simulink model "rolling_contact_36_example"  (R2026b)
settings: Solver=VariableStepAuto  StopTime=5
undefined symbols (not defined in the file): f_rr, k_gx, k_gy, k_x, m_wheel, miu_p, miu_s, mu_slide, mu_stick, omega_rr_eps, r_wheel, sgn, v_gx_max, v_gy_max, vLimit, X, Y, Z
libraries: nesl_utility x225, sm_lib x156, simulink x146, simulink_extras x36
(part 3 of 11)

== system rolling_contact_36_example/36-Point Sliding Contact Model/Body Contact 1 ==
  note: Planar Ground Interaction Model
  " Body Actuator" : nesl_utility/Simulink-PS Converter  PhysicalDomain=network_engine_domain  SubClassName=ps_input  LeftPortType=input  RightPortType=output  PseudoPeriodic=off  Frequencies=[]  NoiseDistribution=none  NoiseParameters=[]  Unit=N  AffineConversion=off  FilteringAndDerivatives=zero  SimscapeFilterOrder=1  InputFilterTimeConstant=.001  UdotUserProvided=0
  " Body Actuator1" : nesl_utility/Simulink-PS Converter  PhysicalDomain=network_engine_domain  SubClassName=ps_input  LeftPortType=input  RightPortType=output  PseudoPeriodic=off  Frequencies=[]  NoiseDistribution=none  NoiseParameters=[]  Unit=N  AffineConversion=off  FilteringAndDerivatives=zero  SimscapeFilterOrder=1  InputFilterTimeConstant=.001  UdotUserProvided=0
  External Force and Torque : sm_lib/Forces and Torques/External Force and Torque  EnableForceX=on  EnableForceY=on  EnableForceZ=off  EnableForce=off  ForceResolutionFrame=World  EnableTorqueX=off  EnableTorqueY=off  EnableTorqueZ=off  EnableTorque=off  TorqueResolutionFrame=AttachedFrame
  Frame Sensor : sm_lib/Frames and Transforms/Transform Sensor  ObservationFrame=World  ExpressedInFrame=World  RotationSequence=XYX  SenseAngle=off  SenseAxis=off  SenseQ=off  SenseR=off  SenseRotationSequence=off  SenseOmegaX=off  SenseOmegaY=off  SenseOmegaZ=off  SenseOmega=off  SenseQDot=off  SenseRDot=off  SenseRotationSequenceDot=off  SenseAlphaX=off  SenseAlphaY=off  SenseAlphaZ=off  SenseAlpha=off  SenseQDDot=off  SenseRDDot=off  SenseX=on  SenseY=on  SenseZ=off  SenseXYZ=off  SenseRad=off  SenseAzim=off  SenseDist=off  SenseInc=off  SenseXDot=on  SenseYDot=on  SenseZDot=off  SenseXYZDot=off  SenseRadDot=off  SenseAzimDot=off  SenseDistDot=off  SenseIncDot=off  SenseXDDot=off  SenseYDDot=off  SenseZDDot=off  SenseXYZDDot=off  SenseRadDDot=off  SenseAzimDDot=off  SenseDistDDot=off  SenseIncDDot=off
  Ground Friction Model : Subsystem
  PS-Simulink Converter : nesl_utility/PS-Simulink Converter  PhysicalDomain=network_engine_domain  SubClassName=ps_output  LeftPortType=input  RightPortType=output  PseudoPeriodic=off  Frequencies=[]  VectorFormat=1-D array  Unit=m  AffineConversion=off
  PS-Simulink Converter1 : nesl_utility/PS-Simulink Converter  PhysicalDomain=network_engine_domain  SubClassName=ps_output  LeftPortType=input  RightPortType=output  PseudoPeriodic=off  Frequencies=[]  VectorFormat=1-D array  Unit=m  AffineConversion=off
  PS-Simulink Converter2 : nesl_utility/PS-Simulink Converter  PhysicalDomain=network_engine_domain  SubClassName=ps_output  LeftPortType=input  RightPortType=output  PseudoPeriodic=off  Frequencies=[]  VectorFormat=1-D array  Unit=m/s  AffineConversion=off
  PS-Simulink Converter3 : nesl_utility/PS-Simulink Converter  PhysicalDomain=network_engine_domain  SubClassName=ps_output  LeftPortType=input  RightPortType=output  PseudoPeriodic=off  Frequencies=[]  VectorFormat=1-D array  Unit=m/s  AffineConversion=off
  Sum : Sum  Inputs=-+|
  Terminator : Terminator
  World Frame : sm_lib/Frames and Transforms/World Frame
  contact sensor : simulink/Logic and Bit Operations/Compare To Zero  relop=<=  OutDataTypeStr=boolean
  yGround : Constant  Value=0
  F : PMIOPort  Side=Left
  Fx patch [N] : Outport
  Fy patch [N] : Outport  Port=2
  wires:
  PS-Simulink Converter2/1 -> Ground Friction Model/4(vx [m/s])
  PS-Simulink Converter/1 -> Ground Friction Model/3(x [m])
  PS-Simulink Converter3/1 -> Ground Friction Model/2(vy [m/s])
  PS-Simulink Converter1/1 -> Sum/2
  Sum/1 -> contact sensor/1, Ground Friction Model/1(dy [m])
  yGround/1 -> Sum/1
  contact sensor/1 -> Ground Friction Model/Enable
  Ground Friction Model/1(Fy_Ground[N]) -> " Body Actuator1"/1, Fy patch [N]/1
  Ground Friction Model/2(Fx_Friction [N]) -> " Body Actuator"/1, Fx patch [N]/1
  Ground Friction Model/3(Stiction!) -> Terminator/1
  connections:
  World Frame/RConn1 -- Frame Sensor/LConn1
  PS-Simulink Converter2/LConn1 -- Frame Sensor/RConn4
  PS-Simulink Converter1/LConn1 -- Frame Sensor/RConn3
  Frame Sensor/RConn2 -- PS-Simulink Converter/LConn1
  PS-Simulink Converter3/LConn1 -- Frame Sensor/RConn5
  External Force and Torque/RConn1 -- Frame Sensor/RConn1 -- F/RConn1
  External Force and Torque/LConn2 -- " Body Actuator1"/RConn1
  External Force and Torque/LConn1 -- " Body Actuator"/RConn1

== system rolling_contact_36_example/36-Point Sliding Contact Model/Body Contact 10 ==
  note: Planar Ground Interaction Model
  " Body Actuator" : nesl_utility/Simulink-PS Converter  PhysicalDomain=network_engine_domain  SubClassName=ps_input  LeftPortType=input  RightPortType=output  PseudoPeriodic=off  Frequencies=[]  NoiseDistribution=none  NoiseParameters=[]  Unit=N  AffineConversion=off  FilteringAndDerivatives=zero  SimscapeFilterOrder=1  InputFilterTimeConstant=.001  UdotUserProvided=0
  " Body Actuator1" : nesl_utility/Simulink-PS Converter  PhysicalDomain=network_engine_domain  SubClassName=ps_input  LeftPortType=input  RightPortType=output  PseudoPeriodic=off  Frequencies=[]  NoiseDistribution=none  NoiseParameters=[]  Unit=N  AffineConversion=off  FilteringAndDerivatives=zero  SimscapeFilterOrder=1  InputFilterTimeConstant=.001  UdotUserProvided=0
  External Force and Torque : sm_lib/Forces and Torques/External Force and Torque  EnableForceX=on  EnableForceY=on  EnableForceZ=off  EnableForce=off  ForceResolutionFrame=World  EnableTorqueX=off  EnableTorqueY=off  EnableTorqueZ=off  EnableTorque=off  TorqueResolutionFrame=AttachedFrame
  Frame Sensor : sm_lib/Frames and Transforms/Transform Sensor  ObservationFrame=World  ExpressedInFrame=World  RotationSequence=XYX  SenseAngle=off  SenseAxis=off  SenseQ=off  SenseR=off  SenseRotationSequence=off  SenseOmegaX=off  SenseOmegaY=off  SenseOmegaZ=off  SenseOmega=off  SenseQDot=off  SenseRDot=off  SenseRotationSequenceDot=off  SenseAlphaX=off  SenseAlphaY=off  SenseAlphaZ=off  SenseAlpha=off  SenseQDDot=off  SenseRDDot=off  SenseX=on  SenseY=on  SenseZ=off  SenseXYZ=off  SenseRad=off  SenseAzim=off  SenseDist=off  SenseInc=off  SenseXDot=on  SenseYDot=on  SenseZDot=off  SenseXYZDot=off  SenseRadDot=off  SenseAzimDot=off  SenseDistDot=off  SenseIncDot=off  SenseXDDot=off  SenseYDDot=off  SenseZDDot=off  SenseXYZDDot=off  SenseRadDDot=off  SenseAzimDDot=off  SenseDistDDot=off  SenseIncDDot=off
  Ground Friction Model : Subsystem
  PS-Simulink Converter : nesl_utility/PS-Simulink Converter  PhysicalDomain=network_engine_domain  SubClassName=ps_output  LeftPortType=input  RightPortType=output  PseudoPeriodic=off  Frequencies=[]  VectorFormat=1-D array  Unit=m  AffineConversion=off
  PS-Simulink Converter1 : nesl_utility/PS-Simulink Converter  PhysicalDomain=network_engine_domain  SubClassName=ps_output  LeftPortType=input  RightPortType=output  PseudoPeriodic=off  Frequencies=[]  VectorFormat=1-D array  Unit=m  AffineConversion=off
  PS-Simulink Converter2 : nesl_utility/PS-Simulink Converter  PhysicalDomain=network_engine_domain  SubClassName=ps_output  LeftPortType=input  RightPortType=output  PseudoPeriodic=off  Frequencies=[]  VectorFormat=1-D array  Unit=m/s  AffineConversion=off
  PS-Simulink Converter3 : nesl_utility/PS-Simulink Converter  PhysicalDomain=network_engine_domain  SubClassName=ps_output  LeftPortType=input  RightPortType=output  PseudoPeriodic=off  Frequencies=[]  VectorFormat=1-D array  Unit=m/s  AffineConversion=off
  Sum : Sum  Inputs=-+|
  Terminator : Terminator
  World Frame : sm_lib/Frames and Transforms/World Frame
  contact sensor : simulink/Logic and Bit Operations/Compare To Zero  relop=<=  OutDataTypeStr=boolean
  yGround : Constant  Value=0
  F : PMIOPort  Side=Left
  Fx patch [N] : Outport
  Fy patch [N] : Outport  Port=2
  wires:
  Ground Friction Model/3(Stiction!) -> Terminator/1
  Ground Friction Model/2(Fx_Friction [N]) -> " Body Actuator"/1, Fx patch [N]/1
  Ground Friction Model/1(Fy_Ground[N]) -> " Body Actuator1"/1, Fy patch [N]/1
  contact sensor/1 -> Ground Friction Model/Enable
  yGround/1 -> Sum/1
  Sum/1 -> Ground Friction Model/1(dy [m]), contact sensor/1
  PS-Simulink Converter1/1 -> Sum/2
  PS-Simulink Converter3/1 -> Ground Friction Model/2(vy [m/s])
  PS-Simulink Converter/1 -> Ground Friction Model/3(x [m])
  PS-Simulink Converter2/1 -> Ground Friction Model/4(vx [m/s])
  connections:
  External Force and Torque/LConn1 -- " Body Actuator"/RConn1
  External Force and Torque/LConn2 -- " Body Actuator1"/RConn1
  F/RConn1 -- Frame Sensor/RConn1 -- External Force and Torque/RConn1
  PS-Simulink Converter3/LConn1 -- Frame Sensor/RConn5
  Frame Sensor/RConn2 -- PS-Simulink Converter/LConn1
  PS-Simulink Converter1/LConn1 -- Frame Sensor/RConn3
  PS-Simulink Converter2/LConn1 -- Frame Sensor/RConn4
  World Frame/RConn1 -- Frame Sensor/LConn1

== system rolling_contact_36_example/36-Point Sliding Contact Model/Body Contact 11 ==
  note: Planar Ground Interaction Model
  " Body Actuator" : nesl_utility/Simulink-PS Converter  PhysicalDomain=network_engine_domain  SubClassName=ps_input  LeftPortType=input  RightPortType=output  PseudoPeriodic=off  Frequencies=[]  NoiseDistribution=none  NoiseParameters=[]  Unit=N  AffineConversion=off  FilteringAndDerivatives=zero  SimscapeFilterOrder=1  InputFilterTimeConstant=.001  UdotUserProvided=0
  " Body Actuator1" : nesl_utility/Simulink-PS Converter  PhysicalDomain=network_engine_domain  SubClassName=ps_input  LeftPortType=input  RightPortType=output  PseudoPeriodic=off  Frequencies=[]  NoiseDistribution=none  NoiseParameters=[]  Unit=N  AffineConversion=off  FilteringAndDerivatives=zero  SimscapeFilterOrder=1  InputFilterTimeConstant=.001  UdotUserProvided=0
  External Force and Torque : sm_lib/Forces and Torques/External Force and Torque  EnableForceX=on  EnableForceY=on  EnableForceZ=off  EnableForce=off  ForceResolutionFrame=World  EnableTorqueX=off  EnableTorqueY=off  EnableTorqueZ=off  EnableTorque=off  TorqueResolutionFrame=AttachedFrame
  Frame Sensor : sm_lib/Frames and Transforms/Transform Sensor  ObservationFrame=World  ExpressedInFrame=World  RotationSequence=XYX  SenseAngle=off  SenseAxis=off  SenseQ=off  SenseR=off  SenseRotationSequence=off  SenseOmegaX=off  SenseOmegaY=off  SenseOmegaZ=off  SenseOmega=off  SenseQDot=off  SenseRDot=off  SenseRotationSequenceDot=off  SenseAlphaX=off  SenseAlphaY=off  SenseAlphaZ=off  SenseAlpha=off  SenseQDDot=off  SenseRDDot=off  SenseX=on  SenseY=on  SenseZ=off  SenseXYZ=off  SenseRad=off  SenseAzim=off  SenseDist=off  SenseInc=off  SenseXDot=on  SenseYDot=on  SenseZDot=off  SenseXYZDot=off  SenseRadDot=off  SenseAzimDot=off  SenseDistDot=off  SenseIncDot=off  SenseXDDot=off  SenseYDDot=off  SenseZDDot=off  SenseXYZDDot=off  SenseRadDDot=off  SenseAzimDDot=off  SenseDistDDot=off  SenseIncDDot=off
  Ground Friction Model : Subsystem
  PS-Simulink Converter : nesl_utility/PS-Simulink Converter  PhysicalDomain=network_engine_domain  SubClassName=ps_output  LeftPortType=input  RightPortType=output  PseudoPeriodic=off  Frequencies=[]  VectorFormat=1-D array  Unit=m  AffineConversion=off
  PS-Simulink Converter1 : nesl_utility/PS-Simulink Converter  PhysicalDomain=network_engine_domain  SubClassName=ps_output  LeftPortType=input  RightPortType=output  PseudoPeriodic=off  Frequencies=[]  VectorFormat=1-D array  Unit=m  AffineConversion=off
  PS-Simulink Converter2 : nesl_utility/PS-Simulink Converter  PhysicalDomain=network_engine_domain  SubClassName=ps_output  LeftPortType=input  RightPortType=output  PseudoPeriodic=off  Frequencies=[]  VectorFormat=1-D array  Unit=m/s  AffineConversion=off
  PS-Simulink Converter3 : nesl_utility/PS-Simulink Converter  PhysicalDomain=network_engine_domain  SubClassName=ps_output  LeftPortType=input  RightPortType=output  PseudoPeriodic=off  Frequencies=[]  VectorFormat=1-D array  Unit=m/s  AffineConversion=off
  Sum : Sum  Inputs=-+|
  Terminator : Terminator
  World Frame : sm_lib/Frames and Transforms/World Frame
  contact sensor : simulink/Logic and Bit Operations/Compare To Zero  relop=<=  OutDataTypeStr=boolean
  yGround : Constant  Value=0
  F : PMIOPort  Side=Left
  Fx patch [N] : Outport
  Fy patch [N] : Outport  Port=2
  wires:
  PS-Simulink Converter2/1 -> Ground Friction Model/4(vx [m/s])
  PS-Simulink Converter/1 -> Ground Friction Model/3(x [m])
  PS-Simulink Converter3/1 -> Ground Friction Model/2(vy [m/s])
  PS-Simulink Converter1/1 -> Sum/2
  Sum/1 -> contact sensor/1, Ground Friction Model/1(dy [m])
  yGround/1 -> Sum/1
  contact sensor/1 -> Ground Friction Model/Enable
  Ground Friction Model/1(Fy_Ground[N]) -> " Body Actuator1"/1, Fy patch [N]/1
  Ground Friction Model/2(Fx_Friction [N]) -> " Body Actuator"/1, Fx patch [N]/1
  Ground Friction Model/3(Stiction!) -> Terminator/1
  connections:
  World Frame/RConn1 -- Frame Sensor/LConn1
  PS-Simulink Converter2/LConn1 -- Frame Sensor/RConn4
  PS-Simulink Converter1/LConn1 -- Frame Sensor/RConn3
  Frame Sensor/RConn2 -- PS-Simulink Converter/LConn1
  PS-Simulink Converter3/LConn1 -- Frame Sensor/RConn5
  External Force and Torque/RConn1 -- Frame Sensor/RConn1 -- F/RConn1
  External Force and Torque/LConn2 -- " Body Actuator1"/RConn1
  External Force and Torque/LConn1 -- " Body Actuator"/RConn1

== system rolling_contact_36_example/36-Point Sliding Contact Model/Body Contact 12 ==
  note: Planar Ground Interaction Model
  " Body Actuator" : nesl_utility/Simulink-PS Converter  PhysicalDomain=network_engine_domain  SubClassName=ps_input  LeftPortType=input  RightPortType=output  PseudoPeriodic=off  Frequencies=[]  NoiseDistribution=none  NoiseParameters=[]  Unit=N  AffineConversion=off  FilteringAndDerivatives=zero  SimscapeFilterOrder=1  InputFilterTimeConstant=.001  UdotUserProvided=0
  " Body Actuator1" : nesl_utility/Simulink-PS Converter  PhysicalDomain=network_engine_domain  SubClassName=ps_input  LeftPortType=input  RightPortType=output  PseudoPeriodic=off  Frequencies=[]  NoiseDistribution=none  NoiseParameters=[]  Unit=N  AffineConversion=off  FilteringAndDerivatives=zero  SimscapeFilterOrder=1  InputFilterTimeConstant=.001  UdotUserProvided=0
  External Force and Torque : sm_lib/Forces and Torques/External Force and Torque  EnableForceX=on  EnableForceY=on  EnableForceZ=off  EnableForce=off  ForceResolutionFrame=World  EnableTorqueX=off  EnableTorqueY=off  EnableTorqueZ=off  EnableTorque=off  TorqueResolutionFrame=AttachedFrame
  Frame Sensor : sm_lib/Frames and Transforms/Transform Sensor  ObservationFrame=World  ExpressedInFrame=World  RotationSequence=XYX  SenseAngle=off  SenseAxis=off  SenseQ=off  SenseR=off  SenseRotationSequence=off  SenseOmegaX=off  SenseOmegaY=off  SenseOmegaZ=off  SenseOmega=off  SenseQDot=off  SenseRDot=off  SenseRotationSequenceDot=off  SenseAlphaX=off  SenseAlphaY=off  SenseAlphaZ=off  SenseAlpha=off  SenseQDDot=off  SenseRDDot=off  SenseX=on  SenseY=on  SenseZ=off  SenseXYZ=off  SenseRad=off  SenseAzim=off  SenseDist=off  SenseInc=off  SenseXDot=on  SenseYDot=on  SenseZDot=off  SenseXYZDot=off  SenseRadDot=off  SenseAzimDot=off  SenseDistDot=off  SenseIncDot=off  SenseXDDot=off  SenseYDDot=off  SenseZDDot=off  SenseXYZDDot=off  SenseRadDDot=off  SenseAzimDDot=off  SenseDistDDot=off  SenseIncDDot=off
  Ground Friction Model : Subsystem
  PS-Simulink Converter : nesl_utility/PS-Simulink Converter  PhysicalDomain=network_engine_domain  SubClassName=ps_output  LeftPortType=input  RightPortType=output  PseudoPeriodic=off  Frequencies=[]  VectorFormat=1-D array  Unit=m  AffineConversion=off
  PS-Simulink Converter1 : nesl_utility/PS-Simulink Converter  PhysicalDomain=network_engine_domain  SubClassName=ps_output  LeftPortType=input  RightPortType=output  PseudoPeriodic=off  Frequencies=[]  VectorFormat=1-D array  Unit=m  AffineConversion=off
  PS-Simulink Converter2 : nesl_utility/PS-Simulink Converter  PhysicalDomain=network_engine_domain  SubClassName=ps_output  LeftPortType=input  RightPortType=output  PseudoPeriodic=off  Frequencies=[]  VectorFormat=1-D array  Unit=m/s  AffineConversion=off
  PS-Simulink Converter3 : nesl_utility/PS-Simulink Converter  PhysicalDomain=network_engine_domain  SubClassName=ps_output  LeftPortType=input  RightPortType=output  PseudoPeriodic=off  Frequencies=[]  VectorFormat=1-D array  Unit=m/s  AffineConversion=off
  Sum : Sum  Inputs=-+|
  Terminator : Terminator
  World Frame : sm_lib/Frames and Transforms/World Frame
  contact sensor : simulink/Logic and Bit Operations/Compare To Zero  relop=<=  OutDataTypeStr=boolean
  yGround : Constant  Value=0
  F : PMIOPort  Side=Left
  Fx patch [N] : Outport
  Fy patch [N] : Outport  Port=2
  wires:
  Ground Friction Model/3(Stiction!) -> Terminator/1
  Ground Friction Model/2(Fx_Friction [N]) -> " Body Actuator"/1, Fx patch [N]/1
  Ground Friction Model/1(Fy_Ground[N]) -> " Body Actuator1"/1, Fy patch [N]/1
  contact sensor/1 -> Ground Friction Model/Enable
  yGround/1 -> Sum/1
  Sum/1 -> Ground Friction Model/1(dy [m]), contact sensor/1
  PS-Simulink Converter1/1 -> Sum/2
  PS-Simulink Converter3/1 -> Ground Friction Model/2(vy [m/s])
  PS-Simulink Converter/1 -> Ground Friction Model/3(x [m])
  PS-Simulink Converter2/1 -> Ground Friction Model/4(vx [m/s])
  connections:
  External Force and Torque/LConn1 -- " Body Actuator"/RConn1
  External Force and Torque/LConn2 -- " Body Actuator1"/RConn1
  F/RConn1 -- Frame Sensor/RConn1 -- External Force and Torque/RConn1
  PS-Simulink Converter3/LConn1 -- Frame Sensor/RConn5
  Frame Sensor/RConn2 -- PS-Simulink Converter/LConn1
  PS-Simulink Converter1/LConn1 -- Frame Sensor/RConn3
  PS-Simulink Converter2/LConn1 -- Frame Sensor/RConn4
  World Frame/RConn1 -- Frame Sensor/LConn1

== system rolling_contact_36_example/36-Point Sliding Contact Model/Body Contact 13 ==
  note: Planar Ground Interaction Model
  " Body Actuator" : nesl_utility/Simulink-PS Converter  PhysicalDomain=network_engine_domain  SubClassName=ps_input  LeftPortType=input  RightPortType=output  PseudoPeriodic=off  Frequencies=[]  NoiseDistribution=none  NoiseParameters=[]  Unit=N  AffineConversion=off  FilteringAndDerivatives=zero  SimscapeFilterOrder=1  InputFilterTimeConstant=.001  UdotUserProvided=0
  " Body Actuator1" : nesl_utility/Simulink-PS Converter  PhysicalDomain=network_engine_domain  SubClassName=ps_input  LeftPortType=input  RightPortType=output  PseudoPeriodic=off  Frequencies=[]  NoiseDistribution=none  NoiseParameters=[]  Unit=N  AffineConversion=off  FilteringAndDerivatives=zero  SimscapeFilterOrder=1  InputFilterTimeConstant=.001  UdotUserProvided=0
  External Force and Torque : sm_lib/Forces and Torques/External Force and Torque  EnableForceX=on  EnableForceY=on  EnableForceZ=off  EnableForce=off  ForceResolutionFrame=World  EnableTorqueX=off  EnableTorqueY=off  EnableTorqueZ=off  EnableTorque=off  TorqueResolutionFrame=AttachedFrame
  Frame Sensor : sm_lib/Frames and Transforms/Transform Sensor  ObservationFrame=World  ExpressedInFrame=World  RotationSequence=XYX  SenseAngle=off  SenseAxis=off  SenseQ=off  SenseR=off  SenseRotationSequence=off  SenseOmegaX=off  SenseOmegaY=off  SenseOmegaZ=off  SenseOmega=off  SenseQDot=off  SenseRDot=off  SenseRotationSequenceDot=off  SenseAlphaX=off  SenseAlphaY=off  SenseAlphaZ=off  SenseAlpha=off  SenseQDDot=off  SenseRDDot=off  SenseX=on  SenseY=on  SenseZ=off  SenseXYZ=off  SenseRad=off  SenseAzim=off  SenseDist=off  SenseInc=off  SenseXDot=on  SenseYDot=on  SenseZDot=off  SenseXYZDot=off  SenseRadDot=off  SenseAzimDot=off  SenseDistDot=off  SenseIncDot=off  SenseXDDot=off  SenseYDDot=off  SenseZDDot=off  SenseXYZDDot=off  SenseRadDDot=off  SenseAzimDDot=off  SenseDistDDot=off  SenseIncDDot=off
  Ground Friction Model : Subsystem
  PS-Simulink Converter : nesl_utility/PS-Simulink Converter  PhysicalDomain=network_engine_domain  SubClassName=ps_output  LeftPortType=input  RightPortType=output  PseudoPeriodic=off  Frequencies=[]  VectorFormat=1-D array  Unit=m  AffineConversion=off
  PS-Simulink Converter1 : nesl_utility/PS-Simulink Converter  PhysicalDomain=network_engine_domain  SubClassName=ps_output  LeftPortType=input  RightPortType=output  PseudoPeriodic=off  Frequencies=[]  VectorFormat=1-D array  Unit=m  AffineConversion=off
  PS-Simulink Converter2 : nesl_utility/PS-Simulink Converter  PhysicalDomain=network_engine_domain  SubClassName=ps_output  LeftPortType=input  RightPortType=output  PseudoPeriodic=off  Frequencies=[]  VectorFormat=1-D array  Unit=m/s  AffineConversion=off
  PS-Simulink Converter3 : nesl_utility/PS-Simulink Converter  PhysicalDomain=network_engine_domain  SubClassName=ps_output  LeftPortType=input  RightPortType=output  PseudoPeriodic=off  Frequencies=[]  VectorFormat=1-D array  Unit=m/s  AffineConversion=off
  Sum : Sum  Inputs=-+|
  Terminator : Terminator
  World Frame : sm_lib/Frames and Transforms/World Frame
  contact sensor : simulink/Logic and Bit Operations/Compare To Zero  relop=<=  OutDataTypeStr=boolean
  yGround : Constant  Value=0
  F : PMIOPort  Side=Left
  Fx patch [N] : Outport
  Fy patch [N] : Outport  Port=2
  wires:
  PS-Simulink Converter2/1 -> Ground Friction Model/4(vx [m/s])
  PS-Simulink Converter/1 -> Ground Friction Model/3(x [m])
  PS-Simulink Converter3/1 -> Ground Friction Model/2(vy [m/s])
  PS-Simulink Converter1/1 -> Sum/2
  Sum/1 -> contact sensor/1, Ground Friction Model/1(dy [m])
  yGround/1 -> Sum/1
  contact sensor/1 -> Ground Friction Model/Enable
  Ground Friction Model/1(Fy_Ground[N]) -> " Body Actuator1"/1, Fy patch [N]/1
  Ground Friction Model/2(Fx_Friction [N]) -> " Body Actuator"/1, Fx patch [N]/1
  Ground Friction Model/3(Stiction!) -> Terminator/1
  connections:
  World Frame/RConn1 -- Frame Sensor/LConn1
  PS-Simulink Converter2/LConn1 -- Frame Sensor/RConn4
  PS-Simulink Converter1/LConn1 -- Frame Sensor/RConn3
  Frame Sensor/RConn2 -- PS-Simulink Converter/LConn1
  PS-Simulink Converter3/LConn1 -- Frame Sensor/RConn5
  External Force and Torque/RConn1 -- Frame Sensor/RConn1 -- F/RConn1
  External Force and Torque/LConn2 -- " Body Actuator1"/RConn1
  External Force and Torque/LConn1 -- " Body Actuator"/RConn1

== system rolling_contact_36_example/36-Point Sliding Contact Model/Body Contact 14 ==
  note: Planar Ground Interaction Model
  " Body Actuator" : nesl_utility/Simulink-PS Converter  PhysicalDomain=network_engine_domain  SubClassName=ps_input  LeftPortType=input  RightPortType=output  PseudoPeriodic=off  Frequencies=[]  NoiseDistribution=none  NoiseParameters=[]  Unit=N  AffineConversion=off  FilteringAndDerivatives=zero  SimscapeFilterOrder=1  InputFilterTimeConstant=.001  UdotUserProvided=0
  " Body Actuator1" : nesl_utility/Simulink-PS Converter  PhysicalDomain=network_engine_domain  SubClassName=ps_input  LeftPortType=input  RightPortType=output  PseudoPeriodic=off  Frequencies=[]  NoiseDistribution=none  NoiseParameters=[]  Unit=N  AffineConversion=off  FilteringAndDerivatives=zero  SimscapeFilterOrder=1  InputFilterTimeConstant=.001  UdotUserProvided=0
  External Force and Torque : sm_lib/Forces and Torques/External Force and Torque  EnableForceX=on  EnableForceY=on  EnableForceZ=off  EnableForce=off  ForceResolutionFrame=World  EnableTorqueX=off  EnableTorqueY=off  EnableTorqueZ=off  EnableTorque=off  TorqueResolutionFrame=AttachedFrame
  Frame Sensor : sm_lib/Frames and Transforms/Transform Sensor  ObservationFrame=World  ExpressedInFrame=World  RotationSequence=XYX  SenseAngle=off  SenseAxis=off  SenseQ=off  SenseR=off  SenseRotationSequence=off  SenseOmegaX=off  SenseOmegaY=off  SenseOmegaZ=off  SenseOmega=off  SenseQDot=off  SenseRDot=off  SenseRotationSequenceDot=off  SenseAlphaX=off  SenseAlphaY=off  SenseAlphaZ=off  SenseAlpha=off  SenseQDDot=off  SenseRDDot=off  SenseX=on  SenseY=on  SenseZ=off  SenseXYZ=off  SenseRad=off  SenseAzim=off  SenseDist=off  SenseInc=off  SenseXDot=on  SenseYDot=on  SenseZDot=off  SenseXYZDot=off  SenseRadDot=off  SenseAzimDot=off  SenseDistDot=off  SenseIncDot=off  SenseXDDot=off  SenseYDDot=off  SenseZDDot=off  SenseXYZDDot=off  SenseRadDDot=off  SenseAzimDDot=off  SenseDistDDot=off  SenseIncDDot=off
  Ground Friction Model : Subsystem
  PS-Simulink Converter : nesl_utility/PS-Simulink Converter  PhysicalDomain=network_engine_domain  SubClassName=ps_output  LeftPortType=input  RightPortType=output  PseudoPeriodic=off  Frequencies=[]  VectorFormat=1-D array  Unit=m  AffineConversion=off
  PS-Simulink Converter1 : nesl_utility/PS-Simulink Converter  PhysicalDomain=network_engine_domain  SubClassName=ps_output  LeftPortType=input  RightPortType=output  PseudoPeriodic=off  Frequencies=[]  VectorFormat=1-D array  Unit=m  AffineConversion=off
  PS-Simulink Converter2 : nesl_utility/PS-Simulink Converter  PhysicalDomain=network_engine_domain  SubClassName=ps_output  LeftPortType=input  RightPortType=output  PseudoPeriodic=off  Frequencies=[]  VectorFormat=1-D array  Unit=m/s  AffineConversion=off
  PS-Simulink Converter3 : nesl_utility/PS-Simulink Converter  PhysicalDomain=network_engine_domain  SubClassName=ps_output  LeftPortType=input  RightPortType=output  PseudoPeriodic=off  Frequencies=[]  VectorFormat=1-D array  Unit=m/s  AffineConversion=off
  Sum : Sum  Inputs=-+|
  Terminator : Terminator
  World Frame : sm_lib/Frames and Transforms/World Frame
  contact sensor : simulink/Logic and Bit Operations/Compare To Zero  relop=<=  OutDataTypeStr=boolean
  yGround : Constant  Value=0
  F : PMIOPort  Side=Left
  Fx patch [N] : Outport
  Fy patch [N] : Outport  Port=2
  wires:
  Ground Friction Model/3(Stiction!) -> Terminator/1
  Ground Friction Model/2(Fx_Friction [N]) -> " Body Actuator"/1, Fx patch [N]/1
  Ground Friction Model/1(Fy_Ground[N]) -> " Body Actuator1"/1, Fy patch [N]/1
  contact sensor/1 -> Ground Friction Model/Enable
  yGround/1 -> Sum/1
  Sum/1 -> Ground Friction Model/1(dy [m]), contact sensor/1
  PS-Simulink Converter1/1 -> Sum/2
  PS-Simulink Converter3/1 -> Ground Friction Model/2(vy [m/s])
  PS-Simulink Converter/1 -> Ground Friction Model/3(x [m])
  PS-Simulink Converter2/1 -> Ground Friction Model/4(vx [m/s])
  connections:
  External Force and Torque/LConn1 -- " Body Actuator"/RConn1
  External Force and Torque/LConn2 -- " Body Actuator1"/RConn1
  F/RConn1 -- Frame Sensor/RConn1 -- External Force and Torque/RConn1
  PS-Simulink Converter3/LConn1 -- Frame Sensor/RConn5
  Frame Sensor/RConn2 -- PS-Simulink Converter/LConn1
  PS-Simulink Converter1/LConn1 -- Frame Sensor/RConn3
  PS-Simulink Converter2/LConn1 -- Frame Sensor/RConn4
  World Frame/RConn1 -- Frame Sensor/LConn1

== system rolling_contact_36_example/36-Point Sliding Contact Model/Body Contact 15 ==
  note: Planar Ground Interaction Model
  " Body Actuator" : nesl_utility/Simulink-PS Converter  PhysicalDomain=network_engine_domain  SubClassName=ps_input  LeftPortType=input  RightPortType=output  PseudoPeriodic=off  Frequencies=[]  NoiseDistribution=none  NoiseParameters=[]  Unit=N  AffineConversion=off  FilteringAndDerivatives=zero  SimscapeFilterOrder=1  InputFilterTimeConstant=.001  UdotUserProvided=0
  " Body Actuator1" : nesl_utility/Simulink-PS Converter  PhysicalDomain=network_engine_domain  SubClassName=ps_input  LeftPortType=input  RightPortType=output  PseudoPeriodic=off  Frequencies=[]  NoiseDistribution=none  NoiseParameters=[]  Unit=N  AffineConversion=off  FilteringAndDerivatives=zero  SimscapeFilterOrder=1  InputFilterTimeConstant=.001  UdotUserProvided=0
  External Force and Torque : sm_lib/Forces and Torques/External Force and Torque  EnableForceX=on  EnableForceY=on  EnableForceZ=off  EnableForce=off  ForceResolutionFrame=World  EnableTorqueX=off  EnableTorqueY=off  EnableTorqueZ=off  EnableTorque=off  TorqueResolutionFrame=AttachedFrame
  Frame Sensor : sm_lib/Frames and Transforms/Transform Sensor  ObservationFrame=World  ExpressedInFrame=World  RotationSequence=XYX  SenseAngle=off  SenseAxis=off  SenseQ=off  SenseR=off  SenseRotationSequence=off  SenseOmegaX=off  SenseOmegaY=off  SenseOmegaZ=off  SenseOmega=off  SenseQDot=off  SenseRDot=off  SenseRotationSequenceDot=off  SenseAlphaX=off  SenseAlphaY=off  SenseAlphaZ=off  SenseAlpha=off  SenseQDDot=off  SenseRDDot=off  SenseX=on  SenseY=on  SenseZ=off  SenseXYZ=off  SenseRad=off  SenseAzim=off  SenseDist=off  SenseInc=off  SenseXDot=on  SenseYDot=on  SenseZDot=off  SenseXYZDot=off  SenseRadDot=off  SenseAzimDot=off  SenseDistDot=off  SenseIncDot=off  SenseXDDot=off  SenseYDDot=off  SenseZDDot=off  SenseXYZDDot=off  SenseRadDDot=off  SenseAzimDDot=off  SenseDistDDot=off  SenseIncDDot=off
  Ground Friction Model : Subsystem
  PS-Simulink Converter : nesl_utility/PS-Simulink Converter  PhysicalDomain=network_engine_domain  SubClassName=ps_output  LeftPortType=input  RightPortType=output  PseudoPeriodic=off  Frequencies=[]  VectorFormat=1-D array  Unit=m  AffineConversion=off
  PS-Simulink Converter1 : nesl_utility/PS-Simulink Converter  PhysicalDomain=network_engine_domain  SubClassName=ps_output  LeftPortType=input  RightPortType=output  PseudoPeriodic=off  Frequencies=[]  VectorFormat=1-D array  Unit=m  AffineConversion=off
  PS-Simulink Converter2 : nesl_utility/PS-Simulink Converter  PhysicalDomain=network_engine_domain  SubClassName=ps_output  LeftPortType=input  RightPortType=output  PseudoPeriodic=off  Frequencies=[]  VectorFormat=1-D array  Unit=m/s  AffineConversion=off
  PS-Simulink Converter3 : nesl_utility/PS-Simulink Converter  PhysicalDomain=network_engine_domain  SubClassName=ps_output  LeftPortType=input  RightPortType=output  PseudoPeriodic=off  Frequencies=[]  VectorFormat=1-D array  Unit=m/s  AffineConversion=off
  Sum : Sum  Inputs=-+|
  Terminator : Terminator
  World Frame : sm_lib/Frames and Transforms/World Frame
  contact sensor : simulink/Logic and Bit Operations/Compare To Zero  relop=<=  OutDataTypeStr=boolean
  yGround : Constant  Value=0
  F : PMIOPort  Side=Left
  Fx patch [N] : Outport
  Fy patch [N] : Outport  Port=2
  wires:
  PS-Simulink Converter2/1 -> Ground Friction Model/4(vx [m/s])
  PS-Simulink Converter/1 -> Ground Friction Model/3(x [m])
  PS-Simulink Converter3/1 -> Ground Friction Model/2(vy [m/s])
  PS-Simulink Converter1/1 -> Sum/2
  Sum/1 -> contact sensor/1, Ground Friction Model/1(dy [m])
  yGround/1 -> Sum/1
  contact sensor/1 -> Ground Friction Model/Enable
  Ground Friction Model/1(Fy_Ground[N]) -> " Body Actuator1"/1, Fy patch [N]/1
  Ground Friction Model/2(Fx_Friction [N]) -> " Body Actuator"/1, Fx patch [N]/1
  Ground Friction Model/3(Stiction!) -> Terminator/1
  connections:
  World Frame/RConn1 -- Frame Sensor/LConn1
  PS-Simulink Converter2/LConn1 -- Frame Sensor/RConn4
  PS-Simulink Converter1/LConn1 -- Frame Sensor/RConn3
  Frame Sensor/RConn2 -- PS-Simulink Converter/LConn1
  PS-Simulink Converter3/LConn1 -- Frame Sensor/RConn5
  External Force and Torque/RConn1 -- Frame Sensor/RConn1 -- F/RConn1
  External Force and Torque/LConn2 -- " Body Actuator1"/RConn1
  External Force and Torque/LConn1 -- " Body Actuator"/RConn1

== system rolling_contact_36_example/36-Point Sliding Contact Model/Body Contact 16 ==
  note: Planar Ground Interaction Model
  " Body Actuator" : nesl_utility/Simulink-PS Converter  PhysicalDomain=network_engine_domain  SubClassName=ps_input  LeftPortType=input  RightPortType=output  PseudoPeriodic=off  Frequencies=[]  NoiseDistribution=none  NoiseParameters=[]  Unit=N  AffineConversion=off  FilteringAndDerivatives=zero  SimscapeFilterOrder=1  InputFilterTimeConstant=.001  UdotUserProvided=0
  " Body Actuator1" : nesl_utility/Simulink-PS Converter  PhysicalDomain=network_engine_domain  SubClassName=ps_input  LeftPortType=input  RightPortType=output  PseudoPeriodic=off  Frequencies=[]  NoiseDistribution=none  NoiseParameters=[]  Unit=N  AffineConversion=off  FilteringAndDerivatives=zero  SimscapeFilterOrder=1  InputFilterTimeConstant=.001  UdotUserProvided=0
  External Force and Torque : sm_lib/Forces and Torques/External Force and Torque  EnableForceX=on  EnableForceY=on  EnableForceZ=off  EnableForce=off  ForceResolutionFrame=World  EnableTorqueX=off  EnableTorqueY=off  EnableTorqueZ=off  EnableTorque=off  TorqueResolutionFrame=AttachedFrame
  Frame Sensor : sm_lib/Frames and Transforms/Transform Sensor  ObservationFrame=World  ExpressedInFrame=World  RotationSequence=XYX  SenseAngle=off  SenseAxis=off  SenseQ=off  SenseR=off  SenseRotationSequence=off  SenseOmegaX=off  SenseOmegaY=off  SenseOmegaZ=off  SenseOmega=off  SenseQDot=off  SenseRDot=off  SenseRotationSequenceDot=off  SenseAlphaX=off  SenseAlphaY=off  SenseAlphaZ=off  SenseAlpha=off  SenseQDDot=off  SenseRDDot=off  SenseX=on  SenseY=on  SenseZ=off  SenseXYZ=off  SenseRad=off  SenseAzim=off  SenseDist=off  SenseInc=off  SenseXDot=on  SenseYDot=on  SenseZDot=off  SenseXYZDot=off  SenseRadDot=off  SenseAzimDot=off  SenseDistDot=off  SenseIncDot=off  SenseXDDot=off  SenseYDDot=off  SenseZDDot=off  SenseXYZDDot=off  SenseRadDDot=off  SenseAzimDDot=off  SenseDistDDot=off  SenseIncDDot=off
  Ground Friction Model : Subsystem
  PS-Simulink Converter : nesl_utility/PS-Simulink Converter  PhysicalDomain=network_engine_domain  SubClassName=ps_output  LeftPortType=input  RightPortType=output  PseudoPeriodic=off  Frequencies=[]  VectorFormat=1-D array  Unit=m  AffineConversion=off
  PS-Simulink Converter1 : nesl_utility/PS-Simulink Converter  PhysicalDomain=network_engine_domain  SubClassName=ps_output  LeftPortType=input  RightPortType=output  PseudoPeriodic=off  Frequencies=[]  VectorFormat=1-D array  Unit=m  AffineConversion=off
  PS-Simulink Converter2 : nesl_utility/PS-Simulink Converter  PhysicalDomain=network_engine_domain  SubClassName=ps_output  LeftPortType=input  RightPortType=output  PseudoPeriodic=off  Frequencies=[]  VectorFormat=1-D array  Unit=m/s  AffineConversion=off
  PS-Simulink Converter3 : nesl_utility/PS-Simulink Converter  PhysicalDomain=network_engine_domain  SubClassName=ps_output  LeftPortType=input  RightPortType=output  PseudoPeriodic=off  Frequencies=[]  VectorFormat=1-D array  Unit=m/s  AffineConversion=off
  Sum : Sum  Inputs=-+|
  Terminator : Terminator
  World Frame : sm_lib/Frames and Transforms/World Frame
  contact sensor : simulink/Logic and Bit Operations/Compare To Zero  relop=<=  OutDataTypeStr=boolean
  yGround : Constant  Value=0
  F : PMIOPort  Side=Left
  Fx patch [N] : Outport
  Fy patch [N] : Outport  Port=2
  wires:
  Ground Friction Model/3(Stiction!) -> Terminator/1
  Ground Friction Model/2(Fx_Friction [N]) -> " Body Actuator"/1, Fx patch [N]/1
  Ground Friction Model/1(Fy_Ground[N]) -> " Body Actuator1"/1, Fy patch [N]/1
  contact sensor/1 -> Ground Friction Model/Enable
  yGround/1 -> Sum/1
  Sum/1 -> Ground Friction Model/1(dy [m]), contact sensor/1
  PS-Simulink Converter1/1 -> Sum/2
  PS-Simulink Converter3/1 -> Ground Friction Model/2(vy [m/s])
  PS-Simulink Converter/1 -> Ground Friction Model/3(x [m])
  PS-Simulink Converter2/1 -> Ground Friction Model/4(vx [m/s])
  connections:
  External Force and Torque/LConn1 -- " Body Actuator"/RConn1
  External Force and Torque/LConn2 -- " Body Actuator1"/RConn1
  F/RConn1 -- Frame Sensor/RConn1 -- External Force and Torque/RConn1
  PS-Simulink Converter3/LConn1 -- Frame Sensor/RConn5
  Frame Sensor/RConn2 -- PS-Simulink Converter/LConn1
  PS-Simulink Converter1/LConn1 -- Frame Sensor/RConn3
  PS-Simulink Converter2/LConn1 -- Frame Sensor/RConn4
  World Frame/RConn1 -- Frame Sensor/LConn1

== system rolling_contact_36_example/36-Point Sliding Contact Model/Body Contact 17 ==
  note: Planar Ground Interaction Model
  " Body Actuator" : nesl_utility/Simulink-PS Converter  PhysicalDomain=network_engine_domain  SubClassName=ps_input  LeftPortType=input  RightPortType=output  PseudoPeriodic=off  Frequencies=[]  NoiseDistribution=none  NoiseParameters=[]  Unit=N  AffineConversion=off  FilteringAndDerivatives=zero  SimscapeFilterOrder=1  InputFilterTimeConstant=.001  UdotUserProvided=0
  " Body Actuator1" : nesl_utility/Simulink-PS Converter  PhysicalDomain=network_engine_domain  SubClassName=ps_input  LeftPortType=input  RightPortType=output  PseudoPeriodic=off  Frequencies=[]  NoiseDistribution=none  NoiseParameters=[]  Unit=N  AffineConversion=off  FilteringAndDerivatives=zero  SimscapeFilterOrder=1  InputFilterTimeConstant=.001  UdotUserProvided=0
  External Force and Torque : sm_lib/Forces and Torques/External Force and Torque  EnableForceX=on  EnableForceY=on  EnableForceZ=off  EnableForce=off  ForceResolutionFrame=World  EnableTorqueX=off  EnableTorqueY=off  EnableTorqueZ=off  EnableTorque=off  TorqueResolutionFrame=AttachedFrame
  Frame Sensor : sm_lib/Frames and Transforms/Transform Sensor  ObservationFrame=World  ExpressedInFrame=World  RotationSequence=XYX  SenseAngle=off  SenseAxis=off  SenseQ=off  SenseR=off  SenseRotationSequence=off  SenseOmegaX=off  SenseOmegaY=off  SenseOmegaZ=off  SenseOmega=off  SenseQDot=off  SenseRDot=off  SenseRotationSequenceDot=off  SenseAlphaX=off  SenseAlphaY=off  SenseAlphaZ=off  SenseAlpha=off  SenseQDDot=off  SenseRDDot=off  SenseX=on  SenseY=on  SenseZ=off  SenseXYZ=off  SenseRad=off  SenseAzim=off  SenseDist=off  SenseInc=off  SenseXDot=on  SenseYDot=on  SenseZDot=off  SenseXYZDot=off  SenseRadDot=off  SenseAzimDot=off  SenseDistDot=off  SenseIncDot=off  SenseXDDot=off  SenseYDDot=off  SenseZDDot=off  SenseXYZDDot=off  SenseRadDDot=off  SenseAzimDDot=off  SenseDistDDot=off  SenseIncDDot=off
  Ground Friction Model : Subsystem
  PS-Simulink Converter : nesl_utility/PS-Simulink Converter  PhysicalDomain=network_engine_domain  SubClassName=ps_output  LeftPortType=input  RightPortType=output  PseudoPeriodic=off  Frequencies=[]  VectorFormat=1-D array  Unit=m  AffineConversion=off
  PS-Simulink Converter1 : nesl_utility/PS-Simulink Converter  PhysicalDomain=network_engine_domain  SubClassName=ps_output  LeftPortType=input  RightPortType=output  PseudoPeriodic=off  Frequencies=[]  VectorFormat=1-D array  Unit=m  AffineConversion=off
  PS-Simulink Converter2 : nesl_utility/PS-Simulink Converter  PhysicalDomain=network_engine_domain  SubClassName=ps_output  LeftPortType=input  RightPortType=output  PseudoPeriodic=off  Frequencies=[]  VectorFormat=1-D array  Unit=m/s  AffineConversion=off
  PS-Simulink Converter3 : nesl_utility/PS-Simulink Converter  PhysicalDomain=network_engine_domain  SubClassName=ps_output  LeftPortType=input  RightPortType=output  PseudoPeriodic=off  Frequencies=[]  VectorFormat=1-D array  Unit=m/s  AffineConversion=off
  Sum : Sum  Inputs=-+|
  Terminator : Terminator
  World Frame : sm_lib/Frames and Transforms/World Frame
  contact sensor : simulink/Logic and Bit Operations/Compare To Zero  relop=<=  OutDataTypeStr=boolean
  yGround : Constant  Value=0
  F : PMIOPort  Side=Left
  Fx patch [N] : Outport
  Fy patch [N] : Outport  Port=2
  wires:
  PS-Simulink Converter2/1 -> Ground Friction Model/4(vx [m/s])
  PS-Simulink Converter/1 -> Ground Friction Model/3(x [m])
  PS-Simulink Converter3/1 -> Ground Friction Model/2(vy [m/s])
  PS-Simulink Converter1/1 -> Sum/2
  Sum/1 -> contact sensor/1, Ground Friction Model/1(dy [m])
  yGround/1 -> Sum/1
  contact sensor/1 -> Ground Friction Model/Enable
  Ground Friction Model/1(Fy_Ground[N]) -> " Body Actuator1"/1, Fy patch [N]/1
  Ground Friction Model/2(Fx_Friction [N]) -> " Body Actuator"/1, Fx patch [N]/1
  Ground Friction Model/3(Stiction!) -> Terminator/1
  connections:
  World Frame/RConn1 -- Frame Sensor/LConn1
  PS-Simulink Converter2/LConn1 -- Frame Sensor/RConn4
  PS-Simulink Converter1/LConn1 -- Frame Sensor/RConn3
  Frame Sensor/RConn2 -- PS-Simulink Converter/LConn1
  PS-Simulink Converter3/LConn1 -- Frame Sensor/RConn5
  External Force and Torque/RConn1 -- Frame Sensor/RConn1 -- F/RConn1
  External Force and Torque/LConn2 -- " Body Actuator1"/RConn1
  External Force and Torque/LConn1 -- " Body Actuator"/RConn1

== system rolling_contact_36_example/36-Point Sliding Contact Model/Body Contact 18 ==
  note: Planar Ground Interaction Model
  " Body Actuator" : nesl_utility/Simulink-PS Converter  PhysicalDomain=network_engine_domain  SubClassName=ps_input  LeftPortType=input  RightPortType=output  PseudoPeriodic=off  Frequencies=[]  NoiseDistribution=none  NoiseParameters=[]  Unit=N  AffineConversion=off  FilteringAndDerivatives=zero  SimscapeFilterOrder=1  InputFilterTimeConstant=.001  UdotUserProvided=0
  " Body Actuator1" : nesl_utility/Simulink-PS Converter  PhysicalDomain=network_engine_domain  SubClassName=ps_input  LeftPortType=input  RightPortType=output  PseudoPeriodic=off  Frequencies=[]  NoiseDistribution=none  NoiseParameters=[]  Unit=N  AffineConversion=off  FilteringAndDerivatives=zero  SimscapeFilterOrder=1  InputFilterTimeConstant=.001  UdotUserProvided=0
  External Force and Torque : sm_lib/Forces and Torques/External Force and Torque  EnableForceX=on  EnableForceY=on  EnableForceZ=off  EnableForce=off  ForceResolutionFrame=World  EnableTorqueX=off  EnableTorqueY=off  EnableTorqueZ=off  EnableTorque=off  TorqueResolutionFrame=AttachedFrame
  Frame Sensor : sm_lib/Frames and Transforms/Transform Sensor  ObservationFrame=World  ExpressedInFrame=World  RotationSequence=XYX  SenseAngle=off  SenseAxis=off  SenseQ=off  SenseR=off  SenseRotationSequence=off  SenseOmegaX=off  SenseOmegaY=off  SenseOmegaZ=off  SenseOmega=off  SenseQDot=off  SenseRDot=off  SenseRotationSequenceDot=off  SenseAlphaX=off  SenseAlphaY=off  SenseAlphaZ=off  SenseAlpha=off  SenseQDDot=off  SenseRDDot=off  SenseX=on  SenseY=on  SenseZ=off  SenseXYZ=off  SenseRad=off  SenseAzim=off  SenseDist=off  SenseInc=off  SenseXDot=on  SenseYDot=on  SenseZDot=off  SenseXYZDot=off  SenseRadDot=off  SenseAzimDot=off  SenseDistDot=off  SenseIncDot=off  SenseXDDot=off  SenseYDDot=off  SenseZDDot=off  SenseXYZDDot=off  SenseRadDDot=off  SenseAzimDDot=off  SenseDistDDot=off  SenseIncDDot=off
  Ground Friction Model : Subsystem
  PS-Simulink Converter : nesl_utility/PS-Simulink Converter  PhysicalDomain=network_engine_domain  SubClassName=ps_output  LeftPortType=input  RightPortType=output  PseudoPeriodic=off  Frequencies=[]  VectorFormat=1-D array  Unit=m  AffineConversion=off
  PS-Simulink Converter1 : nesl_utility/PS-Simulink Converter  PhysicalDomain=network_engine_domain  SubClassName=ps_output  LeftPortType=input  RightPortType=output  PseudoPeriodic=off  Frequencies=[]  VectorFormat=1-D array  Unit=m  AffineConversion=off
  PS-Simulink Converter2 : nesl_utility/PS-Simulink Converter  PhysicalDomain=network_engine_domain  SubClassName=ps_output  LeftPortType=input  RightPortType=output  PseudoPeriodic=off  Frequencies=[]  VectorFormat=1-D array  Unit=m/s  AffineConversion=off
  PS-Simulink Converter3 : nesl_utility/PS-Simulink Converter  PhysicalDomain=network_engine_domain  SubClassName=ps_output  LeftPortType=input  RightPortType=output  PseudoPeriodic=off  Frequencies=[]  VectorFormat=1-D array  Unit=m/s  AffineConversion=off
  Sum : Sum  Inputs=-+|
  Terminator : Terminator
  World Frame : sm_lib/Frames and Transforms/World Frame
  contact sensor : simulink/Logic and Bit Operations/Compare To Zero  relop=<=  OutDataTypeStr=boolean
  yGround : Constant  Value=0
  F : PMIOPort  Side=Left
  Fx patch [N] : Outport
  Fy patch [N] : Outport  Port=2
  wires:
  Ground Friction Model/3(Stiction!) -> Terminator/1
  Ground Friction Model/2(Fx_Friction [N]) -> " Body Actuator"/1, Fx patch [N]/1
  Ground Friction Model/1(Fy_Ground[N]) -> " Body Actuator1"/1, Fy patch [N]/1
  contact sensor/1 -> Ground Friction Model/Enable
  yGround/1 -> Sum/1
  Sum/1 -> Ground Friction Model/1(dy [m]), contact sensor/1
  PS-Simulink Converter1/1 -> Sum/2
  PS-Simulink Converter3/1 -> Ground Friction Model/2(vy [m/s])
  PS-Simulink Converter/1 -> Ground Friction Model/3(x [m])
  PS-Simulink Converter2/1 -> Ground Friction Model/4(vx [m/s])
  connections:
  External Force and Torque/LConn1 -- " Body Actuator"/RConn1
  External Force and Torque/LConn2 -- " Body Actuator1"/RConn1
  F/RConn1 -- Frame Sensor/RConn1 -- External Force and Torque/RConn1
  PS-Simulink Converter3/LConn1 -- Frame Sensor/RConn5
  Frame Sensor/RConn2 -- PS-Simulink Converter/LConn1
  PS-Simulink Converter1/LConn1 -- Frame Sensor/RConn3
  PS-Simulink Converter2/LConn1 -- Frame Sensor/RConn4
  World Frame/RConn1 -- Frame Sensor/LConn1

== system rolling_contact_36_example/36-Point Sliding Contact Model/Body Contact 19 ==
  note: Planar Ground Interaction Model
  " Body Actuator" : nesl_utility/Simulink-PS Converter  PhysicalDomain=network_engine_domain  SubClassName=ps_input  LeftPortType=input  RightPortType=output  PseudoPeriodic=off  Frequencies=[]  NoiseDistribution=none  NoiseParameters=[]  Unit=N  AffineConversion=off  FilteringAndDerivatives=zero  SimscapeFilterOrder=1  InputFilterTimeConstant=.001  UdotUserProvided=0
  " Body Actuator1" : nesl_utility/Simulink-PS Converter  PhysicalDomain=network_engine_domain  SubClassName=ps_input  LeftPortType=input  RightPortType=output  PseudoPeriodic=off  Frequencies=[]  NoiseDistribution=none  NoiseParameters=[]  Unit=N  AffineConversion=off  FilteringAndDerivatives=zero  SimscapeFilterOrder=1  InputFilterTimeConstant=.001  UdotUserProvided=0
  External Force and Torque : sm_lib/Forces and Torques/External Force and Torque  EnableForceX=on  EnableForceY=on  EnableForceZ=off  EnableForce=off  ForceResolutionFrame=World  EnableTorqueX=off  EnableTorqueY=off  EnableTorqueZ=off  EnableTorque=off  TorqueResolutionFrame=AttachedFrame
  Frame Sensor : sm_lib/Frames and Transforms/Transform Sensor  ObservationFrame=World  ExpressedInFrame=World  RotationSequence=XYX  SenseAngle=off  SenseAxis=off  SenseQ=off  SenseR=off  SenseRotationSequence=off  SenseOmegaX=off  SenseOmegaY=off  SenseOmegaZ=off  SenseOmega=off  SenseQDot=off  SenseRDot=off  SenseRotationSequenceDot=off  SenseAlphaX=off  SenseAlphaY=off  SenseAlphaZ=off  SenseAlpha=off  SenseQDDot=off  SenseRDDot=off  SenseX=on  SenseY=on  SenseZ=off  SenseXYZ=off  SenseRad=off  SenseAzim=off  SenseDist=off  SenseInc=off  SenseXDot=on  SenseYDot=on  SenseZDot=off  SenseXYZDot=off  SenseRadDot=off  SenseAzimDot=off  SenseDistDot=off  SenseIncDot=off  SenseXDDot=off  SenseYDDot=off  SenseZDDot=off  SenseXYZDDot=off  SenseRadDDot=off  SenseAzimDDot=off  SenseDistDDot=off  SenseIncDDot=off
  Ground Friction Model : Subsystem
  PS-Simulink Converter : nesl_utility/PS-Simulink Converter  PhysicalDomain=network_engine_domain  SubClassName=ps_output  LeftPortType=input  RightPortType=output  PseudoPeriodic=off  Frequencies=[]  VectorFormat=1-D array  Unit=m  AffineConversion=off
  PS-Simulink Converter1 : nesl_utility/PS-Simulink Converter  PhysicalDomain=network_engine_domain  SubClassName=ps_output  LeftPortType=input  RightPortType=output  PseudoPeriodic=off  Frequencies=[]  VectorFormat=1-D array  Unit=m  AffineConversion=off
  PS-Simulink Converter2 : nesl_utility/PS-Simulink Converter  PhysicalDomain=network_engine_domain  SubClassName=ps_output  LeftPortType=input  RightPortType=output  PseudoPeriodic=off  Frequencies=[]  VectorFormat=1-D array  Unit=m/s  AffineConversion=off
  PS-Simulink Converter3 : nesl_utility/PS-Simulink Converter  PhysicalDomain=network_engine_domain  SubClassName=ps_output  LeftPortType=input  RightPortType=output  PseudoPeriodic=off  Frequencies=[]  VectorFormat=1-D array  Unit=m/s  AffineConversion=off
  Sum : Sum  Inputs=-+|
  Terminator : Terminator
  World Frame : sm_lib/Frames and Transforms/World Frame
  contact sensor : simulink/Logic and Bit Operations/Compare To Zero  relop=<=  OutDataTypeStr=boolean
  yGround : Constant  Value=0
  F : PMIOPort  Side=Left
  Fx patch [N] : Outport
  Fy patch [N] : Outport  Port=2
  wires:
  PS-Simulink Converter2/1 -> Ground Friction Model/4(vx [m/s])
  PS-Simulink Converter/1 -> Ground Friction Model/3(x [m])
  PS-Simulink Converter3/1 -> Ground Friction Model/2(vy [m/s])
  PS-Simulink Converter1/1 -> Sum/2
  Sum/1 -> contact sensor/1, Ground Friction Model/1(dy [m])
  yGround/1 -> Sum/1
  contact sensor/1 -> Ground Friction Model/Enable
  Ground Friction Model/1(Fy_Ground[N]) -> " Body Actuator1"/1, Fy patch [N]/1
  Ground Friction Model/2(Fx_Friction [N]) -> " Body Actuator"/1, Fx patch [N]/1
  Ground Friction Model/3(Stiction!) -> Terminator/1
  connections:
  World Frame/RConn1 -- Frame Sensor/LConn1
  PS-Simulink Converter2/LConn1 -- Frame Sensor/RConn4
  PS-Simulink Converter1/LConn1 -- Frame Sensor/RConn3
  Frame Sensor/RConn2 -- PS-Simulink Converter/LConn1
  PS-Simulink Converter3/LConn1 -- Frame Sensor/RConn5
  External Force and Torque/RConn1 -- Frame Sensor/RConn1 -- F/RConn1
  External Force and Torque/LConn2 -- " Body Actuator1"/RConn1
  External Force and Torque/LConn1 -- " Body Actuator"/RConn1
